simulink model "Task_dcIntroEq_PID"  (R2019b)
settings: Solver=ode45  StartTime=0.0  StopTime=10.0  MaxStep=0.1  RelTol=1e-3  EnableMultiTasking=on
InitFcn:
  | dcMotorParams
values from neighbouring files (symbols this model uses):
  K = 1./R    [velProfCalcFunction.m]
undefined symbols (not defined in the file or in its folder): b, J, L, R
settings Model: DataDictionary=DCM_Intro.sldd  EnableAccessToBaseWorkspace=off  Creator=deastman  LastModifiedBy=valakshe
settings DataIOCC: LimitDataPoints=on  SaveFormat=Array  InspectSignalLogs=on  ReturnWorkspaceOutputs=off
settings OptimizationCC: ExpressionDepthLimit=2147483647  InitFltsAndDblsToZero=on  LifeSpan=inf
settings DebuggingCC: UnderspecifiedInitializationDetection=Classic  MergeDetectMultiDrivingBlocksExec=none  SolverPrmCheckMsg=warning  FcnCallInpInsideContextMsg=warning  StateNameClashWarn=warning  SFUnexpectedBacktrackingDiag=warning  SFNoUnconditionalDefaultTransitionDiag=warning  SFExecutionAtInitializationDiag=none  ArithmeticOperatorsInVariantConditions=warning
settings HardwareCC: ProdBitPerPointer=32  ProdBitPerSizeT=32  ProdBitPerPtrDiffT=32  ProdLargestAtomicFloat=None  ProdIntDivRoundTo=Undefined  ProdEndianess=Unspecified  ProdWordSize=32  ProdHWDeviceType=32-bit Generic
settings ModelReferenceCC: PropagateSignalLabelsOutOfModel=off
settings SFSimCC: SimUseLocalCustomCode=off  CustomCodeUndefinedFunction=UseInterfaceOnly
settings RTWCC: RTWUseLocalCustomCode=off
settings CodeAppCC: StateflowObjectComments=on
settings GRTTargetCC: TargetLangStandard=C89/C90 (ANSI)  GeneratePreprocessorConditionals=Disable all  CombineOutputUpdateFcns=off  GRTInterface=on
settings ConfigComp: CovMetricSettings=dw  CovHtmlReporting=on  CovSaveCumulativeToWorkspaceVar=on  CovSaveSingleToWorkspaceVar=on  CovExternalEMLEnable=off  CovSFcnEnable=off

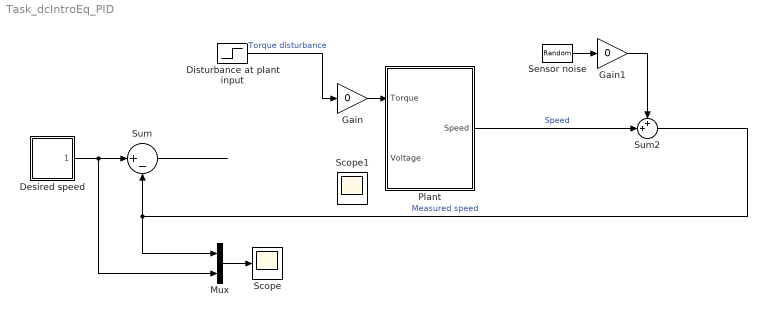
== system Task_dcIntroEq_PID ==
  " Disturbance at plant input" : Step  Time=5  After=0.2  SampleTime=0
  Desired speed : Subsystem
  Gain : Gain  Gain=0
  Gain1 : Gain  Gain=0
  Mux : Mux  Inputs=2
  Plant : Subsystem
  Scope : Scope
  Scope1 : Scope
  Sensor noise : RandomNumber  Variance=0.05  SampleTime=0
  Sum : Sum  Inputs=|+-
  Sum2 : Sum  Inputs=++|
  wires:
  Sum/1 -> ?
  Desired speed/1(Speed) -> Mux/2, Sum/1
  Plant/1(Speed) -> Sum2/2  "Speed"
  Sensor noise/1 -> Gain1/1
  " Disturbance at plant input"/1 -> Gain/1  "Torque disturbance"
  Sum2/1 -> Mux/1, Sum/2  "Measured speed"
  ? -> Scope1/1, Plant/2(Voltage)
  Mux/1 -> Scope/1
  Gain/1 -> Plant/1(Torque)
  Gain1/1 -> Sum2/1

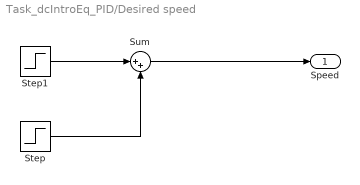
== system Task_dcIntroEq_PID/Desired speed ==
  Step : Step  Time=7  After=-4  SampleTime=0.02
  Step1 : Step  After=2  SampleTime=0.02
  Sum : Sum  Inputs=|++
  Speed : Outport  VectorParamsAs1DForOutWhenUnconnected=off
  wires:
  Step/1 -> Sum/2
  Step1/1 -> Sum/1
  Sum/1 -> Speed/1

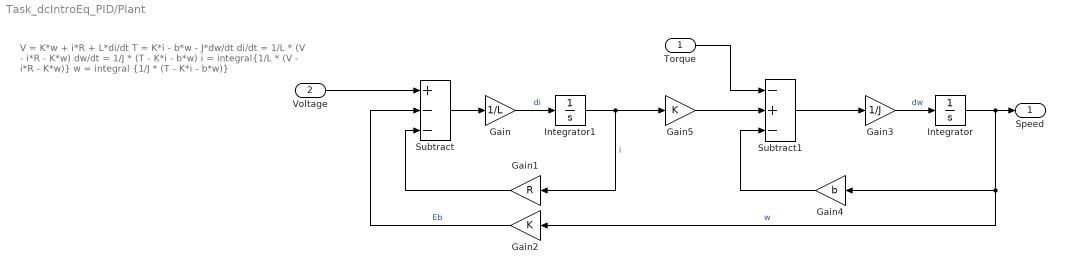
== system Task_dcIntroEq_PID/Plant ==
  note: V = K*w + i*R + L*di/dt
      | T = K*i - b*w - J*dw/dt
      |
      | di/dt = 1/L * (V - i*R - K*w)
      | dw/dt = 1/J * (T - K*i - b*w)
      |
      | i = integral{1/L * (V - i*R - K*w)}
      | w = integral {1/J * (T - K*i - b*w)}
  Torque : Inport
  Voltage : Inport  Port=2
  Gain : Gain  Gain=1/L
  Gain1 : Gain  Gain=R
  Gain2 : Gain  Gain=K
  Gain3 : Gain  Gain=1/J
  Gain4 : Gain  Gain=b
  Gain5 : Gain  Gain=K
  Integrator : Integrator
  Integrator1 : Integrator
  Subtract : Sum  Inputs=+--
  Subtract1 : Sum  Inputs=-+-
  Speed : Outport  VectorParamsAs1DForOutWhenUnconnected=off
  wires:
  Gain/1 -> Integrator1/1  "di"
  Integrator1/1 -> Gain1/1, Gain5/1  "i"
  Subtract/1 -> Gain/1
  Gain1/1 -> Subtract/3
  Gain2/1 -> Subtract/2  "Eb"
  Gain3/1 -> Integrator/1  "dw"
  Subtract1/1 -> Gain3/1
  Integrator/1 -> Gain4/1, Gain2/1, Speed/1  "w"
  Gain5/1 -> Subtract1/2
  Gain4/1 -> Subtract1/3
  Voltage/1 -> Subtract/1
  Torque/1 -> Subtract1/1
